simulink model "jumeau_banc_rw"  (R2025b)
settings: Solver=ode23t  StartTime=0.0  StopTime=20  MaxStep=1e-3  RelTol=1e-4
PostLoadFcn:
  | d = fileparts(get_param('jumeau_banc_rw', 'FileName')); addpath(fullfile(d, 'geometrie'), fullfile(d, 'liaison'), fullfile(d, 'pilotage')); clear d
StartFcn:
  | % Jumeau Webots : au lancement, MATLAB envoie les paramètres du Model Workspace à Webots, qui remet le banc en
  | % position de départ, puis ouvre la liaison de télémétrie et la liaison de commande (liaison/pont_banc.m).
  | if strcmp(get_param('jumeau_banc_rw/Procédé', 'LabelModeActiveChoice'), 'Webots')
  |     pont_banc('ouvrir', getVariable(get_param('jumeau_banc_rw', 'ModelWorkspace'), 'config_jumeau'));
  | end
  | pilotage_banc('depart');   % interface de pilotage : nouveau lancement
StopFcn:
  | pont_banc('fermer');
  | pilotage_banc('fin');
model workspace (MATLAB code in the model file):
  | %% Jumeau numérique du banc de stabilisation à 4 roues de réaction (version 3) : paramètres
  | % Ce code est enregistré dans le modèle (Model Explorer > jumeau_banc_rw > Model Workspace).
  | % Origine : (CAO) CAO du banc version 3, (M) mesuré sur le matériel, (F) fiche technique, (Fw) firmware,
  | % (H) hypothèse à mesurer sur le banc. Masses et inerties des pièces : dans chaque bloc de pièce.
  | 
  | %% Montage de l'essai
  | pivot_mm = 25;              % position du pivot de tangage sur le corps : 25, 24, 16, 8, 0, -8 mm (25 : banc équilibré, rangée +24 et paliers remontés de 1 mm)
  | blocage_roulis = 0;         % goupille de blocage : 1 = axe bloqué à 0°, 0 = axe libre
  | blocage_tangage = 0;
  | angle0_roulis_deg = 2;      % position de départ (mise à 0 si l'axe est bloqué)
  | angle0_tangage_deg = -1;
  | g = 9.81;                   % m/s²
  | 
  | %% Pupitre : pilotage manuel des 4 ESC
  | essai_t = 1;                % s, instant de l'échelon d'essai ajouté aux curseurs
  | essai_echelon_us = [0 0 0 0];   % µs, échelon d'essai sur chaque ESC (0 : aucun)
  | 
  | %% Alimentation des ESC
  | V_alim = 12;                % V, alimentation de labo (H : tension réglée)
  | 
  | %% ESC Brushless 30A bidirectionnels (x4)
  | f_trame_esc = 50;           % Hz, une impulsion toutes les 20 ms (Fw : LEDC 50 Hz)
  | imp_neutre = 1500;          % µs, neutre (testé sur le banc)
  | imp_min = 1000;             % µs (Fw)
  | imp_max = 2000;             % µs (Fw)
  | zone_morte_us = 0;          % µs autour du neutre (H)
  | tau_esc = 2e-3;             % s, temps de réponse de l'ESC (H)
  | armement_actif = 1;         % 1 : l'ESC ne pilote le moteur qu'après t_armement au neutre
  | t_armement = 1;             % s (H)
  | fenetre_armement_us = 25;   % µs, écart au neutre accepté pendant l'armement (H)
  | sens_moteurs = [1 1 1 1];   % +1 : au-dessus du neutre, la roue tourne dans le sens +axe (vers l'extérieur) (H : ordre des phases)
  | 
  | %% Moteurs A2212 1400 KV (x4), modèle équivalent continu
  | KV = 1400;                  % tr/min/V (F)
  | Ke = 60/(2*pi*KV);          % V.s/rad
  | Kt = Ke;                    % N.m/A
  | R_moteur = 0.08;            % ohm (H)
  | L_moteur = 30e-6;           % H (H)
  | f_roue = 5e-6;              % N.m.s/rad, frottement visqueux des roulements du moteur (H)
  | 
  | %% Cardan
  | butee_deg = 20;             % débattement de chaque axe (CAO)
  | k_butee = 20;               % N.m/rad, contact goupille-lumière (H)
  | c_butee = 0.2;              % N.m.s/rad (H)
  | b_cardan = 1e-4;            % N.m.s/rad, frottement des roulements 625 (H)
  | k_cables = 0;               % N.m/rad, raideur des deux câbles vers la table (H)
  | 
  | %% BNO055 (mode fusion)
  | T_bno = 0.01;               % s, données de fusion à 100 Hz (F)
  | bruit_bno = 1;              % 1 : bruit de mesure, 0 : capteur parfait
  | sigma_angle_deg = 0.05;     % ° (H)
  | sigma_gyro_dps = 0.1;       % °/s (H)
  | sigma_acc = 0.02;           % m/s² (H)
  | R_montage_bno = eye(3);     % axes du capteur dans le repère du dispositif : eye(3) = remappage AXIS_MAP réglé
  |                             % (la carte est tournée de 90° dans la CAO)
  | 
  | %% Capteurs de vitesse TCRT5000 (x4) : un front à chaque rayon du disque
  | n_rayons = 4;               % rayons du disque vus par tour (CAO : disque d'origine)
  | T_tcrt = 1e-3;              % s, pas de calcul du capteur (les fronts sont datés par interpolation, comme un chronomètre en µs)
  | t_arret_tcrt = 0.2;         % s sans front : la vitesse mesurée retombe à 0 (Fw, à fixer)
  | 
  | %% Pont vers le jumeau Webots (et, plus tard, vers l'ESP32 du banc réel)
  | T_pont = 0.01;              % s, une trame de commande et une trame de télémétrie toutes les 10 ms
  | 
  | %% Essai : maintien au départ et perturbation
  | t_lacher = 2;                % s, le dispositif est tenu à la main à sa position de départ jusqu'à cet instant (0 : libre dès le départ)
  | k_main = 5;                  % N.m/rad, raideur de la main qui tient le dispositif
  | c_main = 0.3;                % N.m.s/rad, son amortissement
  | perturbation_t = 7;          % s, instant de la poussée d'essai
  | perturbation_duree = 0.2;    % s
  | perturbation_couple = [0.02 0.02];   % N.m, couple de la poussée sur [roulis tangage], programmée (0 : aucune ; l'interface de pilotage en ajoute)
  | 
  | %% Grandeurs dérivées
  | assert(any(pivot_mm == [25 24 16 8 0 -8]), 'pivot_mm : 25, 24, 16, 8, 0, -8');
  | q0_deg = [angle0_roulis_deg angle0_tangage_deg] .* ([blocage_roulis blocage_tangage] == 0);
  | config_jumeau = [pivot_mm; blocage_roulis; blocage_tangage; q0_deg(:); V_alim; f_trame_esc; imp_neutre; imp_min; imp_max; ...
  |     zone_morte_us; tau_esc; armement_actif; t_armement; fenetre_armement_us; sens_moteurs(:); Ke; Kt; R_moteur; L_moteur; ...
  |     f_roue; butee_deg; k_butee; c_butee; b_cardan; k_cables; g; T_bno; bruit_bno; sigma_angle_deg; sigma_gyro_dps; ...
  |     sigma_acc; n_rayons; t_arret_tcrt; T_tcrt; R_montage_bno(:); T_pont; t_lacher; k_main; c_main];   % 51 valeurs envoyées au jumeau Webots au lancement
  | 
  | %% Commande bas niveau : une boucle de vitesse par roue, avec observateur CFO (méthode du TP2, ramenée à la vitesse)
  | J_roue = 1.562e-4;          % kg.m², inertie d'une roue autour de son axe : disque, vis, cloche du moteur (CAO)
  | T_cbn = 1/f_trame_esc;      % s, période de calcul de la commande : celle des ESC, qui ne lisent qu'une impulsion toutes les 20 ms
  | wc_roue = [10 10 10 10];    % rad/s, rapidité du suivi de vitesse de chaque roue (pôle de l'erreur en -wc)
  | wo_roue = [5 5 5 5];        % rad/s, rapidité du CFO de chaque roue (pôles en -wo et -4 wo) ; au-delà de 10, il devient instable à 20 ms
  | imp_cmd_min = 1375;         % µs, limites des impulsions commandées : vitesse conseillée des disques, 3 900 tr/min
  | imp_cmd_max = 1625;         % µs
  | w_aveugle = 45;             % rad/s, en dessous (vitesse du modèle), le TCRT5000 voit mal la roue : le CFO ne se corrige plus sur la mesure
  | 
  | %% Consigne d'essai des roues : ajoutée à la consigne qui vient de la conversion (0 tant qu'elle est vide)
  | essai_roue_t1 = 2;                  % s, départ vers le premier palier
  | essai_roue_vitesse1 = [0 0 0 0];  % rad/s, premier palier de chaque roue (0 : la roue reste à l'arrêt)
  | essai_roue_t2 = 6;                  % s, départ vers le second palier
  | essai_roue_vitesse2 = [0 0 0 0];    % rad/s, second palier de chaque roue
  | essai_roue_acc = 300;               % rad/s², pente des rampes entre les paliers
  | 
  | %% Commande bas niveau : grandeurs calculées
  | % modèle local d'une roue : d(omega)/dt = -a1 omega + a0 V + d
  | a0_roue = Kt/(R_moteur*J_roue) * [1 1 1 1];                % rad/s² par volt
  | a1_roue = (Kt*Ke/R_moteur + f_roue)/J_roue * [1 1 1 1];    % 1/s
  | K_roue = wc_roue - a1_roue;                                % retour d'état : erreur en -(a1 + K) = -wc
  | l1_roue = 5*wo_roue;                                       % CFO
  | lambda_roue = 4/5*wo_roue;
  | 
  | %% Référence : angles demandés au dispositif, en polynômes de degré 5 entre deux paliers
  | ref_t = [2 12];              % s, instant de départ vers chaque palier
  | ref_roulis_deg = [0 5];      % °, roulis demandé à chaque palier
  | ref_tangage_deg = [0 0];     % °, tangage demandé à chaque palier
  | ref_duree = 1.5;             % s, durée du passage d'un palier au suivant
  | 
  | %% Commande haut niveau : une boucle par axe [roulis tangage], placement de pôles basé sur l'observateur CFO (TP2)
  | T_chn = T_cbn;               % s, période de calcul : celle de la commande bas niveau et des ESC
  | t_depart = t_lacher;         % s, mise en marche de la commande : au moment où la main lâche le dispositif
  | wc_axe = [4 4];              % rad/s, rapidité du suivi d'angle de chaque axe
  | xi_axe = [1 1];              % amortissement
  | wo_axe = [3 3];              % rad/s, rapidité du CFO de chaque axe (pôles en -wo et -4 wo, double) ; au-delà de 4, le couple s'agite
  | desat_active = 0;            % 1 : la référence est décalée pour ramener les roues vers leur vitesse de repos
  | T_desat = 5;                 % s, constante de temps de ce retour
  | desat_max_deg = 15;          % °, décalage maximal de la référence
  | 
  | %% Conversion : couples des deux axes vers les 4 roues
  | w_repos = 200;               % rad/s, vitesse de repos des 4 roues : elles tournent toujours, le TCRT5000 les voit toujours
  | t_roues = t_armement + 0.2;  % s, mise en rotation des roues, une fois les ESC armés
  | acc_roue_max = 300;          % rad/s², accélération maximale demandée à une roue
  | w_roue_min = 60;             % rad/s, vitesses limites demandées à une roue
  | w_roue_max = 400;            % rad/s (disques : 3 900 tr/min conseillés, soit 408 rad/s)
  | 
  | %% Masses et inerties utilisées par la commande (CAO du banc version 3)
  | m_disp = 1.2615;             % kg, dispositif et ses 4 roues
  | zG_disp = 24.977e-3;         % m, hauteur de son centre de masse sur le corps (le pivot est à pivot_mm)
  | Ixx_disp_24 = 8.2684e-3;     % kg.m², inertie du dispositif autour du roulis, pivot à +24 mm
  | Iyy_disp_24 = 8.2786e-3;     % kg.m², autour du tangage, pivot à +24 mm
  | m_croix = 0.0755;            % kg, croisillon et paliers (ne tournent qu'en roulis)
  | zG_croix = 0.257e-3;         % m, hauteur de leur centre de masse au-dessus de l'axe de roulis
  | Ixx_croix = 2.073e-4;        % kg.m²
  | 
  | %% Commande haut niveau et conversion : grandeurs calculées
  | % modèle local d'un axe : d²(theta)/dt² = -a1 d(theta)/dt + a0 C + d, avec C le couple demandé aux roues
  | hz = zG_disp - pivot_mm/1000;                                    % m, centre de masse du dispositif au-dessus du pivot
  | I_axe = [Ixx_disp_24 + Ixx_croix, Iyy_disp_24] + m_disp*(hz^2 - (zG_disp - 0.024)^2) - 2*J_roue;   % kg.m²
  | mgh_axe = g*[m_disp*hz + m_croix*zG_croix, m_disp*hz];           % N.m/rad, couple de pesanteur par radian d'inclinaison
  | a0_axe = 1./I_axe;                                               % rad/s² par N.m
  | a1_axe = b_cardan./I_axe;                                        % 1/s
  | k1_axe = wc_axe.^2;                                              % retour d'état : s² + 2 xi wc s + wc²
  | k2_axe = 2*xi_axe.*wc_axe - a1_axe;
  | l1_axe = 9*wo_axe;                                               % CFO du TP2
  | l2_axe = 12*wo_axe.^2;
  | lambda_axe = 4/3*wo_axe;
  | C_max = 2*J_roue*cosd(45)*acc_roue_max;                          % N.m, couple maximal demandé sur un axe
  | k_desat = desat_active.*sign(mgh_axe + (mgh_axe == 0))./(max(abs(mgh_axe), 1e-3)*T_desat);            % rad par N.m.s
  | sx_roues = [1 -1 -1 1];                                          % signe de cos(45°, 135°, 225°, 315°) : part de chaque roue sur le roulis
  | sy_roues = [1 1 -1 -1];                                          % signe de sin : part sur le tangage
  | M_conv = -[sx_roues(:) sy_roues(:)]/(4*J_roue*cosd(45));         % accélération des 4 roues pour un couple [roulis; tangage]
  | 
  | %% Perception : des mesures à l'état du banc
  | T_perception = T_bno;        % s, période de calcul : celle du BNO055
  | tau_desequilibre = 2;        % s, constante de temps du filtre du couple extérieur et du déséquilibre
  | 
  | %% Pilotage par l'interface (pilotage/pilote_banc.m)
  | manche_max_deg = 15;         % °, limite de sécurité de l'inclinaison demandée par le manche (l'interface règle l'amplitude)
  | w_manche = 3;                % rad/s, rapidité avec laquelle la référence rejoint le manche (second ordre critique)
  | T_affichage = 0.1;           % s, rafraîchissement de l'interface
undefined symbols (not defined in the file): DiscIntNeverNeededParam, X, Y, Z
libraries: sm_lib x256, nesl_utility x24, simulink x7
(part 1 of 8)
CloseFcn:
  | try, d = fileparts(get_param('jumeau_banc_rw', 'FileName')); rmpath(fullfile(d, 'geometrie'), fullfile(d, 'liaison'), fullfile(d, 'pilotage')); clear d, catch, end
settings Model: Creator=FOFIEVIGOLBRYAN  LastModifiedBy=FOFIEVIGOLBRYAN

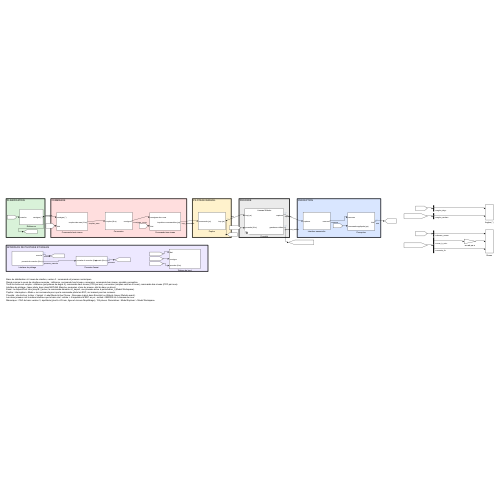
[thumbnail: Simulink's stored preview of the top-level diagram]
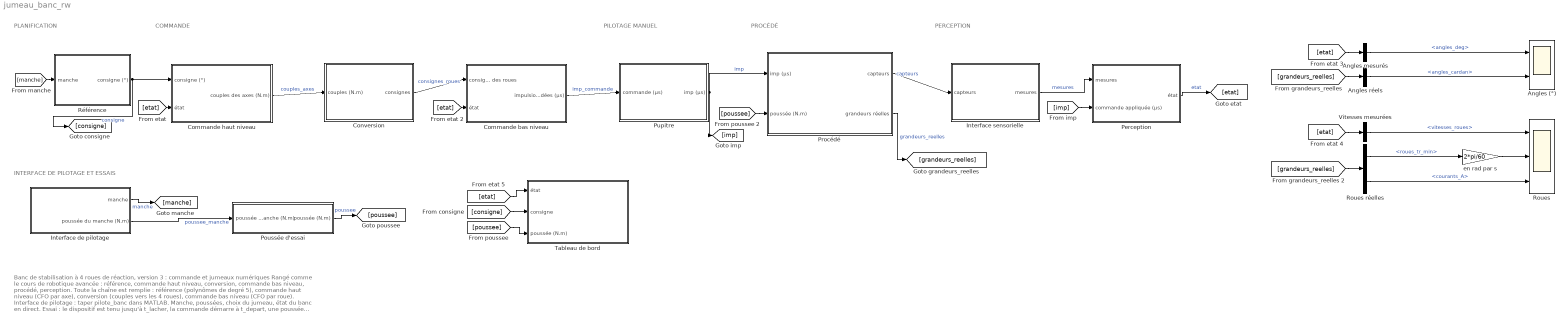
== system jumeau_banc_rw ==
  note: PLANIFICATION
  note: COMMANDE
  note: PILOTAGE MANUEL
  note: PROCÉDÉ
  note: PERCEPTION
  note: Banc de stabilisation à 4 roues de réaction, version 3 : commande et jumeaux numériques
      | Rangé comme le cours de robotique avancée : référence, commande haut niveau, conversion, commande bas niveau, procédé, perception.
      | Toute la chaîne est remplie : référence (polynômes de degré 5), commande haut niveau (CFO par axe), conversion (couples vers les 4 roues), commande bas niveau (CFO par roue).
      | Interface de pilotage : taper pilote_banc dans MATLAB. Manche, poussées, choix du jumeau, état du banc en direct.
      | Essai : le dispositif est tenu jusqu'à t_lacher, la commande démarre à t_depart, une poussée arrive à perturbation_t (Model Workspace).
      | Pupitre : interrupteur « Mode » sur commande pour que la commande pilote les ESC, sur manuel pour les curseurs.
      | Procédé : clic droit sur le bloc > Variant > Label Mode Active Choice : Simscape (calcul dans Simulink) ou Webots (lancer Webots avant).
      | Les deux jumeaux ont la même interface que le banc réel : entrée = 4 impulsions d'ESC en µs ; sorties = BNO055 et 4 vitesses de roue.
      | Mécanique : CAO du banc version 3, équilibrée (pivot à +25 mm, tiges et écrous d'équilibrage), 124 pièces. Paramètres : Model Explorer > Model Workspace.
  note: INTERFACE DE PILOTAGE ET ESSAIS
  Angles (°) : Scope  NumInputPorts=2
      settings: Title=cardan réel : roulis, tangage (°)
  Angles mesurés : BusSelector  OutputSignals=angles_deg
  Angles réels : BusSelector  OutputSignals=angles_cardan
  Commande bas niveau : Subsystem  Description=Commande bas niveau : boucle de vitesse de chaque roue par placement de pôles basé sur l'observateur CFO.
  Commande haut niveau : Subsystem  Description=Commande haut niveau : stabilisation de l'inclinaison par placement de pôles basé sur l'observateur CFO, une boucle par axe.
  Conversion : Subsystem  Description=Conversion : couples des deux axes vers vitesse et accélération de chaque roue.
  Interface de pilotage : Subsystem  Description=Lit le manche et les poussées de l'interface de pilotage.
  Interface sensorielle : Subsystem
  Perception : Subsystem  Description=Perception : des mesures du banc (BNO055, TCRT5000, impulsions envoyées) à son état.
  Poussée d'essai : Subsystem  Description=Poussée d'essai : programmée et demandée par l'interface, envoyée au procédé.
  Procédé : Subsystem  Variant=on  VariantControlMode=label  LabelModeActiveChoice=Webots
  Pupitre : Subsystem
  Roues : Scope  NumInputPorts=3
      settings: ActiveDisplayString=3  Title=courant des moteurs (A)  ActiveDisplayYMinimum=-1  ActiveDisplayYMaximum=1
  Roues réelles : BusSelector  OutputSignals=roues_tr_min,courants_A
  Référence : Subsystem  Description=Référence : angles demandés au dispositif, programmés ou donnés par le manche de l'interface de pilotage.
  Tableau de bord : Subsystem  Description=Tableau de bord : envoie l'état du banc à l'interface de pilotage.
  Vitesses mesurées : BusSelector  OutputSignals=vitesses_roues
  en rad par s : Gain  Gain=2*pi/60
  wires:
  Référence/1(consigne (°)) -> Commande haut niveau/1(consigne (°)), [consigne]  "consigne"
  Commande haut niveau/1(couples des axes (N.m)) -> Conversion/1(couples (N.m))  "couples_axes"
  Conversion/1(consignes) -> Commande bas niveau/1(consignes des roues)  "consignes_roues"
  Commande bas niveau/1(impulsions commandées (µs)) -> Pupitre/1(commande (µs))  "imp_commande"
  Pupitre/1(imp (µs)) -> Procédé/1(imp (µs)), [imp]  "imp"
  Procédé/1(capteurs) -> Interface sensorielle/1(capteurs)  "capteurs"
  Interface sensorielle/1(mesures) -> Perception/1(mesures)  "mesures"
  Perception/1(état) -> [etat]  "etat"
  [etat] -> Commande haut niveau/2(état)
  [etat] -> Commande bas niveau/2(état)
  Procédé/2(grandeurs réelles) -> [grandeurs_reelles]  "grandeurs_reelles"
  [etat] -> Angles mesurés/1
  [grandeurs_reelles] -> Angles réels/1
  [etat] -> Vitesses mesurées/1
  [grandeurs_reelles] -> Roues réelles/1
  Angles mesurés/1 -> Angles (°)/1  "<angles_deg>"
  Angles réels/1 -> Angles (°)/2  "<angles_cardan>"
  Vitesses mesurées/1 -> Roues/1  "<vitesses_roues>"
  Roues réelles/1 -> en rad par s/1  "<roues_tr_min>"
  en rad par s/1 -> Roues/2
  Roues réelles/2 -> Roues/3  "<courants_A>"
  [imp] -> Perception/2(commande appliquée (µs))
  [manche] -> Référence/1(manche)
  Interface de pilotage/1(manche) -> [manche]  "manche"
  Interface de pilotage/2(poussée du manche (N.m)) -> Poussée d'essai/1(poussée du manche (N.m))  "poussee_manche"
  Poussée d'essai/1(poussée (N.m)) -> [poussee]  "poussee"
  [etat] -> Tableau de bord/1(état)
  [consigne] -> Tableau de bord/2(consigne)
  [poussee] -> Tableau de bord/3(poussée (N.m))
  [poussee] -> Procédé/2(poussée (N.m))

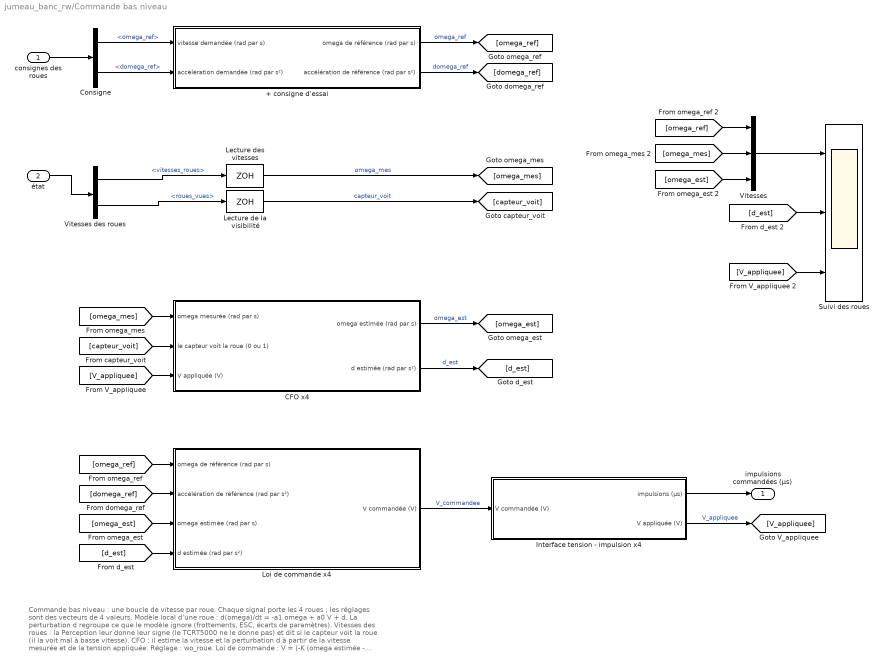
== system jumeau_banc_rw/Commande bas niveau ==
  note: Commande bas niveau : une boucle de vitesse par roue. Chaque signal porte les 4 roues ; les réglages sont des vecteurs de 4 valeurs.
      | Modèle local d'une roue : d(omega)/dt = -a1 omega + a0 V + d. La perturbation d regroupe ce que le modèle ignore (frottements, ESC, écarts de paramètres).
      | Vitesses des roues : la Perception leur donne leur signe (le TCRT5000 ne le donne pas) et dit si le capteur voit la roue (il la voit mal à basse vitesse).
      | CFO : il estime la vitesse et la perturbation d à partir de la vitesse mesurée et de la tension appliquée. Réglage : wo_roue.
      | Loi de commande : V = (-K (omega estimée - omega de référence) - d estimée + a1 omega de référence + accélération de référence) / a0. Réglage : wc_roue.
      | Interface : la tension devient une impulsion d'ESC, bornée de imp_cmd_min à imp_cmd_max. Le CFO reçoit la tension réellement appliquée.
      | Consigne d'essai : essai_roue_... dans le Model Workspace. Pour que la commande pilote les ESC : interrupteur « Mode » du Pupitre sur commande.
  consignes des roues : Inport
  état : Inport  Port=2
  + consigne d'essai : Subsystem
  CFO x4 : Subsystem
  Consigne : BusSelector  OutputSignals=omega_ref,domega_ref
  Interface tension - impulsion x4 : Subsystem
  Lecture de la visibilité : ZeroOrderHold  SampleTime=T_cbn
  Lecture des vitesses : ZeroOrderHold  SampleTime=T_cbn
  Loi de commande x4 : Subsystem
  Suivi des roues : Scope  NumInputPorts=3
      settings: ActiveDisplayString=3  Title=tension appliquée aux moteurs (V)
  Vitesses : Mux  Inputs=3
  Vitesses des roues : BusSelector  OutputSignals=vitesses_roues,roues_vues
  impulsions commandées (µs) : Outport
  wires:
  consignes des roues/1 -> Consigne/1
  Consigne/1 -> + consigne d'essai/1(vitesse demandée (rad par s))  "<omega_ref>"
  Consigne/2 -> + consigne d'essai/2(accélération demandée (rad par s²))  "<domega_ref>"
  + consigne d'essai/1(omega de référence (rad par s)) -> [omega_ref]  "omega_ref"
  + consigne d'essai/2(accélération de référence (rad par s²)) -> [domega_ref]  "domega_ref"
  état/1 -> Vitesses des roues/1
  Vitesses des roues/1 -> Lecture des vitesses/1  "<vitesses_roues>"
  Vitesses des roues/2 -> Lecture de la visibilité/1  "<roues_vues>"
  Lecture des vitesses/1 -> [omega_mes]  "omega_mes"
  Lecture de la visibilité/1 -> [capteur_voit]  "capteur_voit"
  [omega_mes] -> CFO x4/1(omega mesurée (rad par s))
  [capteur_voit] -> CFO x4/2(le capteur voit la roue (0 ou 1))
  [V_appliquee] -> CFO x4/3(V appliquée (V))
  CFO x4/1(omega estimée (rad par s)) -> [omega_est]  "omega_est"
  CFO x4/2(d estimée (rad par s²)) -> [d_est]  "d_est"
  [omega_ref] -> Loi de commande x4/1(omega de référence (rad par s))
  [domega_ref] -> Loi de commande x4/2(accélération de référence (rad par s²))
  [omega_est] -> Loi de commande x4/3(omega estimée (rad par s))
  [d_est] -> Loi de commande x4/4(d estimée (rad par s²))
  Loi de commande x4/1(V commandée (V)) -> Interface tension - impulsion x4/1(V commandée (V))  "V_commandee"
  Interface tension - impulsion x4/1(impulsions (µs)) -> impulsions commandées (µs)/1
  Interface tension - impulsion x4/2(V appliquée (V)) -> [V_appliquee]  "V_appliquee"
  [omega_ref] -> Vitesses/1
  [omega_mes] -> Vitesses/2
  [omega_est] -> Vitesses/3
  Vitesses/1 -> Suivi des roues/1
  [d_est] -> Suivi des roues/2
  [V_appliquee] -> Suivi des roues/3

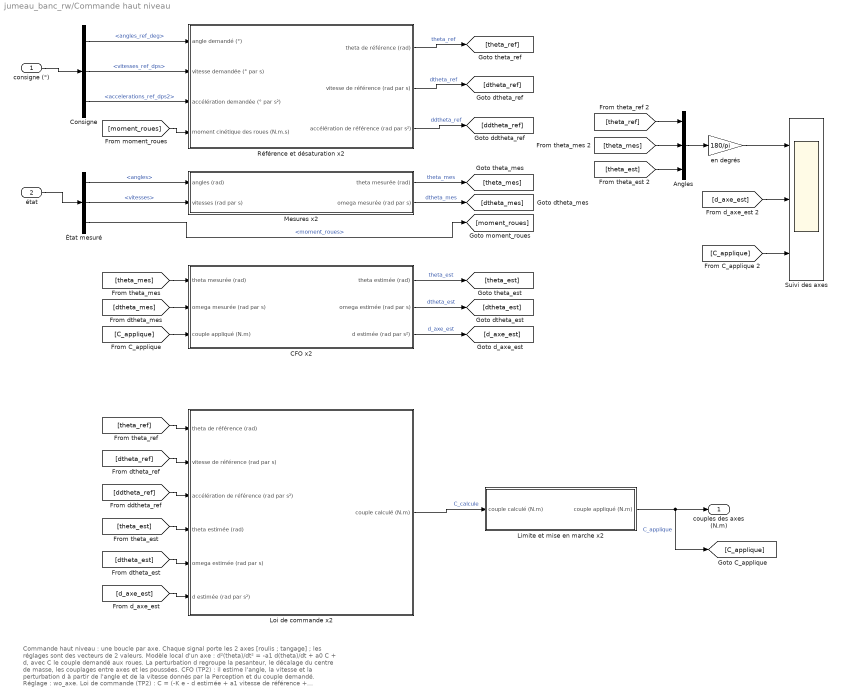
== system jumeau_banc_rw/Commande haut niveau ==
  note: Commande haut niveau : une boucle par axe. Chaque signal porte les 2 axes [roulis ; tangage] ; les réglages sont des vecteurs de 2 valeurs.
      | Modèle local d'un axe : d²(theta)/dt² = -a1 d(theta)/dt + a0 C + d, avec C le couple demandé aux roues. La perturbation d regroupe la pesanteur,
      | le décalage du centre de masse, les couplages entre axes et les poussées.
      | CFO (TP2) : il estime l'angle, la vitesse et la perturbation d à partir de l'angle et de la vitesse donnés par la Perception et du couple demandé. Réglage : wo_axe.
      | Loi de commande (TP2) : C = (-K e - d estimée + a1 vitesse de référence + accélération de référence) / a0. Réglages : wc_axe, xi_axe.
      | Désaturation : la référence est décalée pour que la pesanteur ramène les roues à leur vitesse de repos. Réglages : desat_active, T_desat.
      | La commande démarre à t_depart, quand la main lâche le dispositif. Le couple est borné à C_max.
  consigne (°) : Inport
  état : Inport  Port=2
  Angles : Mux  Inputs=3
  CFO x2 : Subsystem
  Consigne : BusSelector  OutputSignals=angles_ref_deg,vitesses_ref_dps,accelerations_ref_dps2
  Limite et mise en marche x2 : Subsystem
  Loi de commande x2 : Subsystem
  Mesures x2 : Subsystem
  Référence et désaturation x2 : Subsystem
  Suivi des axes : Scope  NumInputPorts=3
      settings: ActiveDisplayString=3  Title=couples demandés aux roues (N.m)
  en degrés : Gain  Gain=180/pi
  État mesuré : BusSelector  OutputSignals=angles,vitesses,moment_roues
  couples des axes (N.m) : Outport
  wires:
  consigne (°)/1 -> Consigne/1
  Consigne/1 -> Référence et désaturation x2/1(angle demandé (°))  "<angles_ref_deg>"
  Consigne/2 -> Référence et désaturation x2/2(vitesse demandée (° par s))  "<vitesses_ref_dps>"
  Consigne/3 -> Référence et désaturation x2/3(accélération demandée (° par s²))  "<accelerations_ref_dps2>"
  [moment_roues] -> Référence et désaturation x2/4(moment cinétique des roues (N.m.s))
  Référence et désaturation x2/1(theta de référence (rad)) -> [theta_ref]  "theta_ref"
  Référence et désaturation x2/2(vitesse de référence (rad par s)) -> [dtheta_ref]  "dtheta_ref"
  Référence et désaturation x2/3(accélération de référence (rad par s²)) -> [ddtheta_ref]  "ddtheta_ref"
  état/1 -> État mesuré/1
  État mesuré/1 -> Mesures x2/1(angles (rad))  "<angles>"
  État mesuré/2 -> Mesures x2/2(vitesses (rad par s))  "<vitesses>"
  État mesuré/3 -> [moment_roues]  "<moment_roues>"
  Mesures x2/1(theta mesurée (rad)) -> [theta_mes]  "theta_mes"
  Mesures x2/2(omega mesurée (rad par s)) -> [dtheta_mes]  "dtheta_mes"
  [theta_mes] -> CFO x2/1(theta mesurée (rad))
  [dtheta_mes] -> CFO x2/2(omega mesurée (rad par s))
  [C_applique] -> CFO x2/3(couple appliqué (N.m))
  CFO x2/1(theta estimée (rad)) -> [theta_est]  "theta_est"
  CFO x2/2(omega estimée (rad par s)) -> [dtheta_est]  "dtheta_est"
  CFO x2/3(d estimée (rad par s²)) -> [d_axe_est]  "d_axe_est"
  [theta_ref] -> Loi de commande x2/1(theta de référence (rad))
  [dtheta_ref] -> Loi de commande x2/2(vitesse de référence (rad par s))
  [ddtheta_ref] -> Loi de commande x2/3(accélération de référence (rad par s²))
  [theta_est] -> Loi de commande x2/4(theta estimée (rad))
  [dtheta_est] -> Loi de commande x2/5(omega estimée (rad par s))
  [d_axe_est] -> Loi de commande x2/6(d estimée (rad par s²))
  Loi de commande x2/1(couple calculé (N.m)) -> Limite et mise en marche x2/1(couple calculé (N.m))  "C_calcule"
  Limite et mise en marche x2/1(couple appliqué (N.m)) -> couples des axes (N.m)/1, [C_applique]  "C_applique"
  [theta_ref] -> Angles/1
  [theta_mes] -> Angles/2
  [theta_est] -> Angles/3
  Angles/1 -> en degrés/1
  en degrés/1 -> Suivi des axes/1
  [d_axe_est] -> Suivi des axes/2
  [C_applique] -> Suivi des axes/3

== system jumeau_banc_rw/Conversion ==
  note: Conversion : couples demandés sur les deux axes vers la vitesse et l'accélération de chaque roue.
      | Une roue qui accélère pousse le dispositif en sens inverse : accélération des 4 roues = M_conv [couple de roulis ; couple de tangage].
      | Les roues sont à 45°, 135°, 225° et 315° : chacune agit sur les deux axes, à part égale (cos 45°).
      | L'accélération s'ajoute à la vitesse de repos w_repos, la même pour les 4 roues : deux roues opposées tournent alors en sens contraire
      | et leurs effets s'annulent. Les roues ne passent jamais par l'arrêt, où le TCRT5000 ne les voit plus.
      | Limites : acc_roue_max sur l'accélération, w_roue_min et w_roue_max sur la vitesse demandée.
  couples (N.m) : Inport
  Accélération demandée : Sum
  Accélération maximale : Saturate  UpperLimit=acc_roue_max  LowerLimit=-acc_roue_max
  Consignes : BusCreator  Description=omega_ref : vitesse demandée à chaque roue (rad/s). domega_ref : son accélération (rad/s²).  Inputs=2
  Mise en rotation : Step  Time=t_roues  Before=[0; 0; 0; 0]  After=w_repos*[1; 1; 1; 1]  SampleTime=T_chn
  Pente de la rampe : simulink/Discrete/Discrete Derivative  gainval=1.0  ICPrevScaledInput=0.0  OutMin=[]  OutMax=[]  OutDataType=fixdt(1, 16)  OutScaling=2^-10  DoSatur=off
  Rampe : RateLimiter  RisingSlewLimit=acc_roue_max  FallingSlewLimit=-acc_roue_max  SampleTimeMode=inherited
  Répartition sur les 4 roues : Gain  Gain=M_conv  Multiplication=Matrix(K*u)
  Vitesse demandée : Sum
  Écart à la vitesse de repos : DiscreteIntegrator  gainval=1  SampleTime=T_chn  LimitOutput=on  UpperSaturationLimit=max(w_roue_max - w_repos, 0)  LowerSaturationLimit=min(w_roue_min - w_repos, 0)  ICPrevOutput=DiscIntNeverNeededParam  ICPrevScaledInput=DiscIntNeverNeededParam
  consignes : Outport
  wires:
  couples (N.m)/1 -> Répartition sur les 4 roues/1
  Répartition sur les 4 roues/1 -> Accélération maximale/1
  Accélération maximale/1 -> [acceleration]  "acceleration"
  [acceleration] -> Écart à la vitesse de repos/1
  Écart à la vitesse de repos/1 -> [ecart_vitesse]  "ecart_vitesse"
  Mise en rotation/1 -> Rampe/1
  Rampe/1 -> [vitesse_repos], Pente de la rampe/1  "vitesse_repos"
  Pente de la rampe/1 -> [acceleration_repos]  "acceleration_repos"
  [ecart_vitesse] -> Vitesse demandée/1
  [vitesse_repos] -> Vitesse demandée/2
  [acceleration] -> Accélération demandée/1
  [acceleration_repos] -> Accélération demandée/2
  Vitesse demandée/1 -> Consignes/1  "omega_ref"
  Accélération demandée/1 -> Consignes/2  "domega_ref"
  Consignes/1 -> consignes/1

== system jumeau_banc_rw/Interface de pilotage ==
  note: Lit l'interface de pilotage (pilotage/pilote_banc.m, échange par pilotage/pilotage_banc.m) à chaque période de la commande.
      | manche = [actif ; roulis demandé ; tangage demandé] (°) ; poussée en cours sur [roulis ; tangage] (N.m).
      | Interface fermée : le manche est inactif (la référence programmée s'applique) et il n'y a aucune poussée.
  Lecture de l'interface : MATLAB Function  TreatAsAtomicUnit=on
  Temps : DigitalClock  SampleTime=T_chn
  manche : Outport
  poussée du manche (N.m) : Outport  Port=2
  wires:
  Temps/1 -> Lecture de l'interface/1(t)
  Lecture de l'interface/1(manche) -> manche/1
  Lecture de l'interface/2(poussee) -> poussée du manche (N.m)/1

== system jumeau_banc_rw/Interface sensorielle ==
  note: Interface sensorielle : ce que l'ESP32 lit sur les capteurs, mis en grandeurs utiles.
      | BNO055 : euler = [cap ; roulis ; tangage] en degrés, gyroscope en °/s. TCRT5000 : vitesse de chaque roue, sans signe.
  note: Quaternion : l'orientation du capteur, au pas de 2^-14. La Perception en tire des angles 8 fois plus fins que les angles d'Euler.
  capteurs : Inport
  Gyroscope : SignalConversion  OverrideOpt=off
  Mesures : BusCreator  Description=angles_deg = [roulis; tangage] (°, angles d'Euler), gyro_dps (°/s, axes du capteur), vitesses_roues (rad/s, sans signe), quaternion [w; x; y; z] (orientation du capteur).  Inputs=4
  Quaternion : SignalConversion  OverrideOpt=off
  Registres lus : BusSelector  OutputSignals=BNO055.euler,BNO055.gyro,vitesses_roues,BNO055.quat
  "Roulis, tangage" : Selector  InputPortWidth=3  IndexOptions=Index vector (dialog)  Indices=[2 3]  OutputSizes=1
  mesures : Outport
  wires:
  capteurs/1 -> Registres lus/1
  Registres lus/1 -> "Roulis, tangage"/1  "<euler>"
  "Roulis, tangage"/1 -> Mesures/1  "angles_deg"
  Registres lus/2 -> Gyroscope/1  "<gyro>"
  Gyroscope/1 -> Mesures/2  "gyro_dps"
  Registres lus/3 -> Mesures/3  "<vitesses_roues>"
  Mesures/1 -> mesures/1
  Registres lus/4 -> Quaternion/1  "<quat>"
  Quaternion/1 -> Mesures/4  "quaternion"

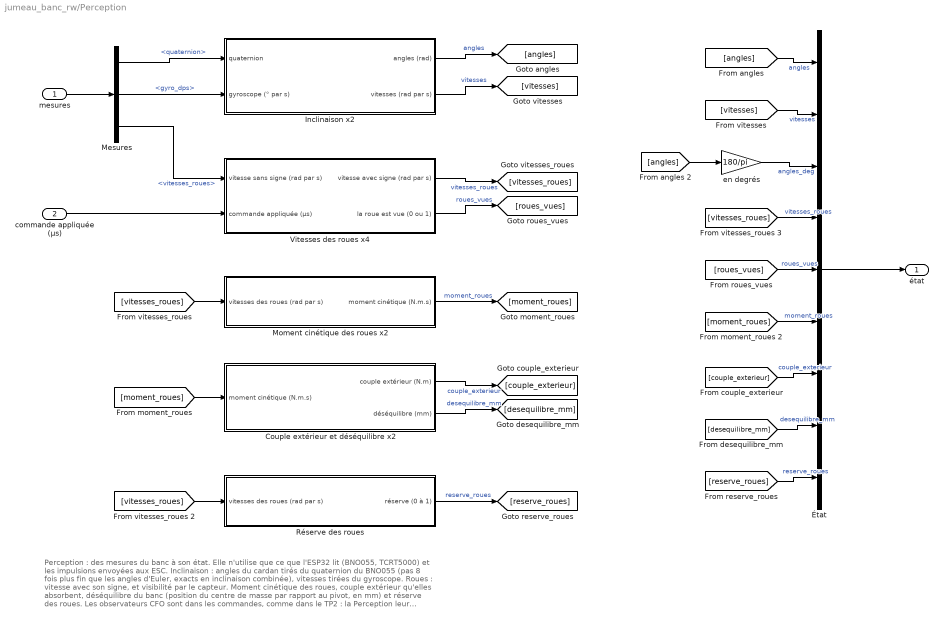
== system jumeau_banc_rw/Perception ==
  note: Perception : des mesures du banc à son état. Elle n'utilise que ce que l'ESP32 lit (BNO055, TCRT5000) et les impulsions envoyées aux ESC.
      | Inclinaison : angles du cardan tirés du quaternion du BNO055 (pas 8 fois plus fin que les angles d'Euler, exacts en inclinaison combinée),
      | vitesses tirées du gyroscope. Roues : vitesse avec son signe, et visibilité par le capteur. Moment cinétique des roues, couple extérieur
      | qu'elles absorbent, déséquilibre du banc (position du centre de masse par rapport au pivot, en mm) et réserve des roues.
      | Les observateurs CFO sont dans les commandes, comme dans le TP2 : la Perception leur donne des mesures propres.
  mesures : Inport
  commande appliquée (µs) : Inport  Port=2
  Couple extérieur et déséquilibre x2 : Subsystem
  Inclinaison x2 : Subsystem
  Mesures : BusSelector  OutputSignals=quaternion,gyro_dps,vitesses_roues
  Moment cinétique des roues x2 : Subsystem
  Réserve des roues : Subsystem
  Vitesses des roues x4 : Subsystem
  en degrés : Gain  Gain=180/pi
  État : BusCreator  Description=angles (rad) et angles_deg (°) : [roulis ; tangage] du cardan ; vitesses (rad/s) ; vitesses_roues (rad/s, avec signe) ; roues_vues (0 ou 1) ; moment_roues (N.m.s, sur [roulis ; tangage]) ; couple_exterieur (N.m) ; desequilibre_mm : position du centre de masse par rapport au pivot, [selon X ; selon Y] ; reserve_roues (0 à 1).  Inputs=9
  état : Outport
  wires:
  mesures/1 -> Mesures/1
  Mesures/1 -> Inclinaison x2/1(quaternion)  "<quaternion>"
  Mesures/2 -> Inclinaison x2/2(gyroscope (° par s))  "<gyro_dps>"
  Inclinaison x2/1(angles (rad)) -> [angles]  "angles"
  Inclinaison x2/2(vitesses (rad par s)) -> [vitesses]  "vitesses"
  Mesures/3 -> Vitesses des roues x4/1(vitesse sans signe (rad par s))  "<vitesses_roues>"
  commande appliquée (µs)/1 -> Vitesses des roues x4/2(commande appliquée (µs))
  Vitesses des roues x4/1(vitesse avec signe (rad par s)) -> [vitesses_roues]  "vitesses_roues"
  Vitesses des roues x4/2(la roue est vue (0 ou 1)) -> [roues_vues]  "roues_vues"
  [vitesses_roues] -> Moment cinétique des roues x2/1(vitesses des roues (rad par s))
  Moment cinétique des roues x2/1(moment cinétique (N.m.s)) -> [moment_roues]  "moment_roues"
  [moment_roues] -> Couple extérieur et déséquilibre x2/1(moment cinétique (N.m.s))
  Couple extérieur et déséquilibre x2/1(couple extérieur (N.m)) -> [couple_exterieur]  "couple_exterieur"
  Couple extérieur et déséquilibre x2/2(déséquilibre (mm)) -> [desequilibre_mm]  "desequilibre_mm"
  [vitesses_roues] -> Réserve des roues/1(vitesses des roues (rad par s))
  Réserve des roues/1(réserve (0 à 1)) -> [reserve_roues]  "reserve_roues"
  [angles] -> État/1  "angles"
  [vitesses] -> État/2  "vitesses"
  [angles] -> en degrés/1
  en degrés/1 -> État/3  "angles_deg"
  [vitesses_roues] -> État/4  "vitesses_roues"
  [roues_vues] -> État/5  "roues_vues"
  [moment_roues] -> État/6  "moment_roues"
  [couple_exterieur] -> État/7  "couple_exterieur"
  [desequilibre_mm] -> État/8  "desequilibre_mm"
  [reserve_roues] -> État/9  "reserve_roues"
  État/1 -> état/1

== system jumeau_banc_rw/Poussée d'essai ==
  note: Poussée sur [roulis ; tangage] (N.m), envoyée au procédé : la poussée programmée (perturbation_t, perturbation_duree,
      | perturbation_couple) plus les poussées demandées par l'interface de pilotage. Le banc réel l'ignorera : on le pousse avec le doigt.
  poussée du manche (N.m) : Inport
  Début de la poussée programmée : Step  Time=perturbation_t  Before=[0; 0]  After=perturbation_couple(:)  SampleTime=0
  Fin de la poussée programmée : Step  Time=perturbation_t + perturbation_duree  Before=[0; 0]  After=-perturbation_couple(:)  SampleTime=0
  Poussée : Sum  Inputs=+++
  poussée (N.m) : Outport
  wires:
  Début de la poussée programmée/1 -> Poussée/1
  Fin de la poussée programmée/1 -> Poussée/2
  poussée du manche (N.m)/1 -> Poussée/3
  Poussée/1 -> poussée (N.m)/1

== system jumeau_banc_rw/Procédé ==
  note: 1) Add Subsystem or Model blocks as valid variant choices.
      | 2) You cannot connect blocks at this level. At simulation, connectivity is automatically
      | determined, based on the active variant and port name matching.
  imp (µs) : Inport
  poussée (N.m) : Inport  Port=2
  Jumeau Simscape : Subsystem  VariantControl=Simscape
  Jumeau Webots : Subsystem  VariantControl=Webots
  capteurs : Outport
  grandeurs réelles : Outport  Port=2

== system jumeau_banc_rw/Pupitre ==
  note: Pupitre : pilotage manuel des 4 ESC, en attendant la commande.
      | Double-clic sur un curseur ESC k : impulsion de 1300 à 1700 µs (1500 = neutre). Les ESC s'arment après 1 s au neutre.
      | Échelon d'essai : essai_echelon_us (Model Workspace) s'ajoute aux curseurs à t = essai_t, pour des essais reproductibles.
      | Double-clic sur un interrupteur pour le basculer : manuel ou commande ; marche ou arrêt (neutre).
  commande (µs) : Inport
  Curseurs : Mux
  Curseurs + essai : Sum
  ESC 1 (µs) : simulink/Math Operations/Slider Gain  gain=1500  low=1300  high=1700
  ESC 2 (µs) : simulink/Math Operations/Slider Gain  gain=1500  low=1300  high=1700
  ESC 3 (µs) : simulink/Math Operations/Slider Gain  gain=1500  low=1300  high=1700
  ESC 4 (µs) : simulink/Math Operations/Slider Gain  gain=1500  low=1300  high=1700
  Marche (haut) ou arrêt (bas) : ManualSwitch
  "Mode : manuel (haut) ou commande (bas)" : ManualSwitch  CurrentSetting=0
  Neutre : Constant  Value=imp_neutre * [1; 1; 1; 1]
  un : Constant
  Échelon d'essai : Step  Time=essai_t  Before=[0; 0; 0; 0]  After=essai_echelon_us(:)  SampleTime=0
  imp (µs) : Outport
  wires:
  un/1 -> ESC 3 (µs)/1, ESC 4 (µs)/1, ESC 1 (µs)/1, ESC 2 (µs)/1
  ESC 1 (µs)/1 -> Curseurs/1
  ESC 2 (µs)/1 -> Curseurs/2
  ESC 3 (µs)/1 -> Curseurs/3
  ESC 4 (µs)/1 -> Curseurs/4
  Curseurs/1 -> Curseurs + essai/1
  Échelon d'essai/1 -> Curseurs + essai/2
  commande (µs)/1 -> [commande]  "commande"
  Curseurs + essai/1 -> "Mode : manuel (haut) ou commande (bas)"/1
  [commande] -> "Mode : manuel (haut) ou commande (bas)"/2
  "Mode : manuel (haut) ou commande (bas)"/1 -> Marche (haut) ou arrêt (bas)/1
  Neutre/1 -> Marche (haut) ou arrêt (bas)/2
  Marche (haut) ou arrêt (bas)/1 -> imp (µs)/1

== system jumeau_banc_rw/Référence ==
  note: Référence : angles de roulis et de tangage demandés au dispositif, avec leur vitesse et leur accélération.
      | Programme : à chaque instant ref_t(i), départ vers le palier [ref_roulis_deg(i) ; ref_tangage_deg(i)], atteint en ref_duree par un polynôme de degré 5.
      | Manche : quand l'interface de pilotage (pilotage/pilote_banc.m) est ouverte, l'angle vient du manche, suivi par un second ordre critique (w_manche).
      | Réglages dans le Model Workspace : ref_t, ref_roulis_deg, ref_tangage_deg, ref_duree, w_manche, manche_max_deg.
  manche : Inport
  "Choix : accélération" : Switch  Criteria=u2 > Threshold  Threshold=0.5  SaturateOnIntegerOverflow=off  InputSameDT=off
  "Choix : angle" : Switch  Criteria=u2 > Threshold  Threshold=0.5  SaturateOnIntegerOverflow=off  InputSameDT=off
  "Choix : vitesse" : Switch  Criteria=u2 > Threshold  Threshold=0.5  SaturateOnIntegerOverflow=off  InputSameDT=off
  Consigne : BusCreator  Description=angles_ref_deg (°), vitesses_ref_dps (°/s), accelerations_ref_dps2 (°/s²), [roulis ; tangage].  Inputs=3
  "Manche : filtre du second ordre" : MATLAB Function  TreatAsAtomicUnit=on
  "Programme : polynômes de degré 5" : MATLAB Function  TreatAsAtomicUnit=on
  Temps : DigitalClock  SampleTime=T_chn
  consigne (°) : Outport
  wires:
  Temps/1 -> "Programme : polynômes de degré 5"/1(t), "Manche : filtre du second ordre"/3(t)
  manche/1 -> "Manche : filtre du second ordre"/1(manche)
  "Programme : polynômes de degré 5"/1(angle) -> "Manche : filtre du second ordre"/2(angle_programme), "Choix : angle"/3
  [manche_actif] -> "Choix : angle"/2
  [manche_actif] -> "Choix : vitesse"/2
  [manche_actif] -> "Choix : accélération"/2
  "Manche : filtre du second ordre"/4(actif) -> [manche_actif]  "manche_actif"
  "Manche : filtre du second ordre"/1(angle) -> "Choix : angle"/1
  "Manche : filtre du second ordre"/2(vitesse) -> "Choix : vitesse"/1
  "Programme : polynômes de degré 5"/2(vitesse) -> "Choix : vitesse"/3
  "Manche : filtre du second ordre"/3(acceleration) -> "Choix : accélération"/1
  "Programme : polynômes de degré 5"/3(acceleration) -> "Choix : accélération"/3
  "Choix : angle"/1 -> Consigne/1  "angles_ref_deg"
  "Choix : vitesse"/1 -> Consigne/2  "vitesses_ref_dps"
  "Choix : accélération"/1 -> Consigne/3  "accelerations_ref_dps2"
  Consigne/1 -> consigne (°)/1

== system jumeau_banc_rw/Tableau de bord ==
  note: Tableau de bord : l'état du banc envoyé à l'interface de pilotage toutes les T_affichage secondes (0,1 s).
      | Il n'utilise que l'état donné par la Perception : il marchera de la même façon avec le banc réel.
  état : Inport
  consigne : Inport  Port=2
  poussée (N.m) : Inport  Port=3
  Consigne : BusSelector  OutputSignals=angles_ref_deg
  Envoi à l'interface : MATLAB Function  TreatAsAtomicUnit=on
  Temps : DigitalClock  SampleTime=T_affichage
  État : BusSelector  OutputSignals=angles_deg,vitesses_roues,reserve_roues,desequilibre_mm
  wires:
  état/1 -> État/1
  consigne/1 -> Consigne/1
  État/1 -> Envoi à l'interface/1(angles_deg)  "<angles_deg>"
  État/2 -> Envoi à l'interface/2(roues)  "<vitesses_roues>"
  État/3 -> Envoi à l'interface/3(reserve)  "<reserve_roues>"
  État/4 -> Envoi à l'interface/4(desequilibre_mm)  "<desequilibre_mm>"
  Consigne/1 -> Envoi à l'interface/5(reference_deg)  "<angles_ref_deg>"
  poussée (N.m)/1 -> Envoi à l'interface/6(poussee)
  Temps/1 -> Envoi à l'interface/7(t)

== system jumeau_banc_rw/Commande bas niveau/+ consigne d'essai ==
  note: Consigne d'essai, ajoutée à la consigne qui vient de la conversion : deux paliers de vitesse reliés par des rampes.
      | Réglages dans le Model Workspace : essai_roue_t1, essai_roue_vitesse1, essai_roue_t2, essai_roue_vitesse2, essai_roue_acc.
      | La pente de la rampe donne l'accélération de référence. Pour ne rien ajouter : mettre les deux paliers à [0 0 0 0].
  vitesse demandée (rad par s) : Inport
  accélération demandée (rad par s²) : Inport  Port=2
  + accélération d'essai : Sum
  + vitesse d'essai : Sum
  Lecture de l'accélération : ZeroOrderHold  SampleTime=T_cbn
  Lecture de la vitesse : ZeroOrderHold  SampleTime=T_cbn
  Palier 1 : Step  Time=essai_roue_t1  Before=[0; 0; 0; 0]  After=essai_roue_vitesse1(:)  SampleTime=T_cbn
  Palier 2 : Step  Time=essai_roue_t2  Before=[0; 0; 0; 0]  After=essai_roue_vitesse2(:) - essai_roue_vitesse1(:)  SampleTime=T_cbn
  Paliers : Sum
  Pente de la rampe : simulink/Discrete/Discrete Derivative  gainval=1.0  ICPrevScaledInput=0.0  OutMin=[]  OutMax=[]  OutDataType=fixdt(1, 16)  OutScaling=2^-10  DoSatur=off
  Rampe : RateLimiter  RisingSlewLimit=essai_roue_acc  FallingSlewLimit=-essai_roue_acc  SampleTimeMode=inherited
  omega de référence (rad par s) : Outport
  accélération de référence (rad par s²) : Outport  Port=2
  wires:
  vitesse demandée (rad par s)/1 -> Lecture de la vitesse/1
  accélération demandée (rad par s²)/1 -> Lecture de l'accélération/1
  Lecture de la vitesse/1 -> + vitesse d'essai/1
  Lecture de l'accélération/1 -> + accélération d'essai/1
  [vitesse_essai] -> + vitesse d'essai/2
  [acceleration_essai] -> + accélération d'essai/2
  + vitesse d'essai/1 -> omega de référence (rad par s)/1
  + accélération d'essai/1 -> accélération de référence (rad par s²)/1
  Palier 1/1 -> Paliers/1
  Palier 2/1 -> Paliers/2
  Paliers/1 -> Rampe/1
  Rampe/1 -> [vitesse_essai], Pente de la rampe/1  "vitesse_essai"
  Pente de la rampe/1 -> [acceleration_essai]  "acceleration_essai"

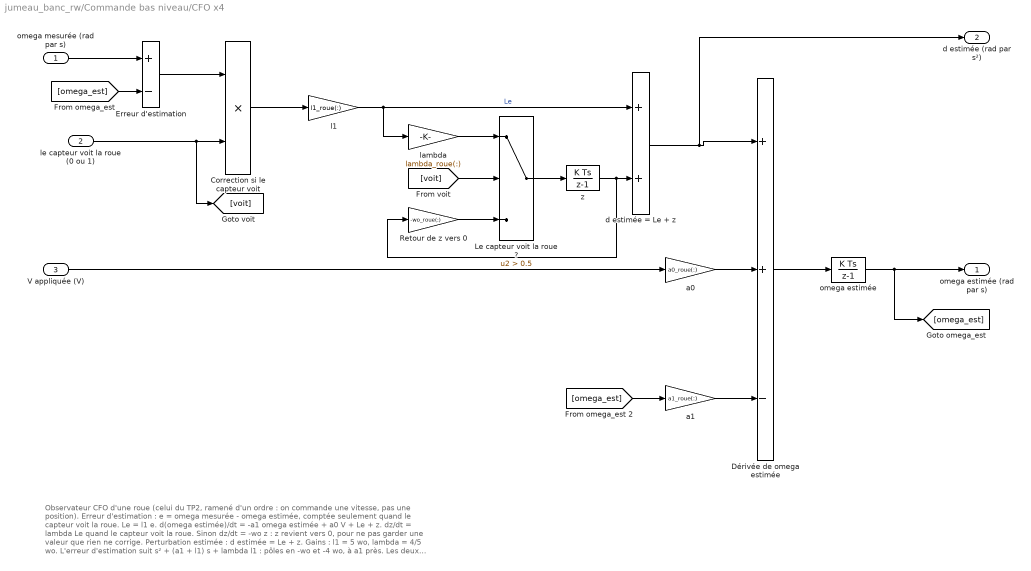
== system jumeau_banc_rw/Commande bas niveau/CFO x4 ==
  note: Observateur CFO d'une roue (celui du TP2, ramené d'un ordre : on commande une vitesse, pas une position).
      | Erreur d'estimation : e = omega mesurée - omega estimée, comptée seulement quand le capteur voit la roue.          Le = l1 e.
      | d(omega estimée)/dt = -a1 omega estimée + a0 V + Le + z.
      | dz/dt = lambda Le quand le capteur voit la roue. Sinon dz/dt = -wo z : z revient vers 0, pour ne pas garder une valeur que rien ne corrige.
      | Perturbation estimée : d estimée = Le + z.
      | Gains : l1 = 5 wo, lambda = 4/5 wo. L'erreur d'estimation suit s² + (a1 + l1) s + lambda l1 : pôles en -wo et -4 wo, à a1 près.
      | Les deux intégrateurs sont discrets (Euler, période T_cbn).
  omega mesurée (rad par s) : Inport
  le capteur voit la roue (0 ou 1) : Inport  Port=2
  V appliquée (V) : Inport  Port=3
  Correction si le capteur voit : Product
  Dérivée de omega estimée : Sum  Inputs=++-
  Erreur d'estimation : Sum  Inputs=+-
  Le capteur voit la roue ? : Switch  Criteria=u2 > Threshold  Threshold=0.5  SaturateOnIntegerOverflow=off  InputSameDT=off
  Retour de z vers 0 : Gain  Gain=-wo_roue(:)
  a0 : Gain  Gain=a0_roue(:)
  a1 : Gain  Gain=a1_roue(:)
  d estimée = Le + z : Sum
  l1 : Gain  Gain=l1_roue(:)
  lambda : Gain  Gain=lambda_roue(:)
  omega estimée : DiscreteIntegrator  gainval=1  SampleTime=T_cbn  ICPrevOutput=DiscIntNeverNeededParam  ICPrevScaledInput=DiscIntNeverNeededParam
  z : DiscreteIntegrator  gainval=1  SampleTime=T_cbn  ICPrevOutput=DiscIntNeverNeededParam  ICPrevScaledInput=DiscIntNeverNeededParam
  omega estimée (rad par s) : Outport
  d estimée (rad par s²) : Outport  Port=2
  wires:
  omega mesurée (rad par s)/1 -> Erreur d'estimation/1
  [omega_est] -> Erreur d'estimation/2
  Erreur d'estimation/1 -> Correction si le capteur voit/1
  le capteur voit la roue (0 ou 1)/1 -> Correction si le capteur voit/2, [voit]
  Correction si le capteur voit/1 -> l1/1
  l1/1 -> d estimée = Le + z/1, lambda/1  "Le"
  lambda/1 -> Le capteur voit la roue ?/1
  [voit] -> Le capteur voit la roue ?/2
  Retour de z vers 0/1 -> Le capteur voit la roue ?/3
  Le capteur voit la roue ?/1 -> z/1
  z/1 -> d estimée = Le + z/2, Retour de z vers 0/1
  d estimée = Le + z/1 -> Dérivée de omega estimée/1, d estimée (rad par s²)/1
  V appliquée (V)/1 -> a0/1
  a0/1 -> Dérivée de omega estimée/2
  [omega_est] -> a1/1
  a1/1 -> Dérivée de omega estimée/3
  Dérivée de omega estimée/1 -> omega estimée/1
  omega estimée/1 -> omega estimée (rad par s)/1, [omega_est]

== system jumeau_banc_rw/Commande bas niveau/Interface tension - impulsion x4 ==
  note: Interface tension - impulsion : l'ESC applique V = V_alim (impulsion - neutre) / (imp_max - imp_neutre), dans le sens de rotation du moteur.
      | L'impulsion est bornée de imp_cmd_min à imp_cmd_max (vitesse conseillée des disques) et arrondie à 1 µs, comme dans la trame de commande.
      | Seconde sortie : la tension réellement appliquée, recalculée à partir de l'impulsion envoyée. C'est elle que le CFO doit recevoir.
  V commandée (V) : Inport
  + neutre : Bias  Bias=imp_neutre  SaturateOnIntegerOverflow=off
  - neutre : Bias  Bias=-imp_neutre  SaturateOnIntegerOverflow=off
  Arrondi à 1 µs : Rounding  Operator=round
  Limites des disques : Saturate  UpperLimit=imp_cmd_max  LowerLimit=imp_cmd_min
  Sens de rotation : Gain  Gain=sens_moteurs(:)
  Sens de rotation (retour) : Gain  Gain=sens_moteurs(:)
  Volts vers µs : Gain  Gain=(imp_max - imp_neutre)/V_alim
  µs vers volts : Gain  Gain=V_alim/(imp_max - imp_neutre)
  impulsions (µs) : Outport
  V appliquée (V) : Outport  Port=2
  wires:
  V commandée (V)/1 -> Volts vers µs/1
  Volts vers µs/1 -> Sens de rotation/1
  Sens de rotation/1 -> + neutre/1
  + neutre/1 -> Limites des disques/1
  Limites des disques/1 -> Arrondi à 1 µs/1
  Arrondi à 1 µs/1 -> impulsions (µs)/1, [impulsions]
  [impulsions] -> - neutre/1
  - neutre/1 -> Sens de rotation (retour)/1
  Sens de rotation (retour)/1 -> µs vers volts/1
  µs vers volts/1 -> V appliquée (V)/1

== system jumeau_banc_rw/Commande bas niveau/Loi de commande x4 ==
  note: Loi de commande d'une roue (celle du TP2, ramenée à la vitesse).
      | Erreur de suivi : e = omega estimée - omega de référence. Commande virtuelle : -K e, avec K = wc - a1. L'erreur suit alors de/dt = -wc e.
      | Tension : V = (-K e - d estimée + a1 omega de référence + accélération de référence) / a0.
  omega de référence (rad par s) : Inport
  accélération de référence (rad par s²) : Inport  Port=2
  omega estimée (rad par s) : Inport  Port=3
  d estimée (rad par s²) : Inport  Port=4
  1 sur a0 : Gain  Gain=1./a0_roue(:)
  Erreur de suivi : Sum  Inputs=+-
  K : Gain  Gain=K_roue(:)
  Somme : Sum  Inputs=++--
  a1 : Gain  Gain=a1_roue(:)
  V commandée (V) : Outport
  wires:
  omega de référence (rad par s)/1 -> a1/1, [omega_ref]
  a1/1 -> Somme/1
  accélération de référence (rad par s²)/1 -> Somme/2
  omega estimée (rad par s)/1 -> Erreur de suivi/1
  [omega_ref] -> Erreur de suivi/2
  Erreur de suivi/1 -> K/1
  K/1 -> Somme/3
  d estimée (rad par s²)/1 -> Somme/4
  Somme/1 -> 1 sur a0/1
  1 sur a0/1 -> V commandée (V)/1

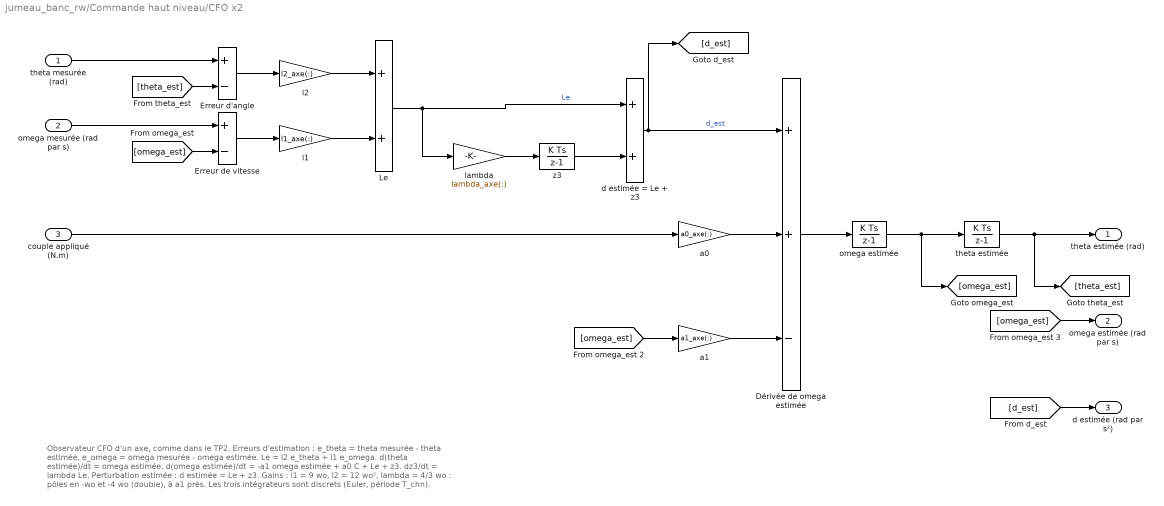
== system jumeau_banc_rw/Commande haut niveau/CFO x2 ==
  note: Observateur CFO d'un axe, comme dans le TP2.
      | Erreurs d'estimation : e_theta = theta mesurée - theta estimée, e_omega = omega mesurée - omega estimée.          Le = l2 e_theta + l1 e_omega.
      | d(theta estimée)/dt = omega estimée.
      | d(omega estimée)/dt = -a1 omega estimée + a0 C + Le + z3.
      | dz3/dt = lambda Le.
      | Perturbation estimée : d estimée = Le + z3.
      | Gains : l1 = 9 wo, l2 = 12 wo², lambda = 4/3 wo : pôles en -wo et -4 wo (double), à a1 près.
      | Les trois intégrateurs sont discrets (Euler, période T_chn).
  theta mesurée (rad) : Inport
  omega mesurée (rad par s) : Inport  Port=2
  couple appliqué (N.m) : Inport  Port=3
  Dérivée de omega estimée : Sum  Inputs=++-
  Erreur d'angle : Sum  Inputs=+-
  Erreur de vitesse : Sum  Inputs=+-
  Le : Sum
  a0 : Gain  Gain=a0_axe(:)
  a1 : Gain  Gain=a1_axe(:)
  d estimée = Le + z3 : Sum
  l1 : Gain  Gain=l1_axe(:)
  l2 : Gain  Gain=l2_axe(:)
  lambda : Gain  Gain=lambda_axe(:)
  omega estimée : DiscreteIntegrator  gainval=1  SampleTime=T_chn  ICPrevOutput=DiscIntNeverNeededParam  ICPrevScaledInput=DiscIntNeverNeededParam
  theta estimée : DiscreteIntegrator  gainval=1  InitialCondition=q0_deg(:)*pi/180  SampleTime=T_chn  ICPrevOutput=DiscIntNeverNeededParam  ICPrevScaledInput=DiscIntNeverNeededParam
  z3 : DiscreteIntegrator  gainval=1  SampleTime=T_chn  ICPrevOutput=DiscIntNeverNeededParam  ICPrevScaledInput=DiscIntNeverNeededParam
  theta estimée (rad) : Outport
  omega estimée (rad par s) : Outport  Port=2
  d estimée (rad par s²) : Outport  Port=3
  wires:
  theta mesurée (rad)/1 -> Erreur d'angle/1
  [theta_est] -> Erreur d'angle/2
  omega mesurée (rad par s)/1 -> Erreur de vitesse/1
  [omega_est] -> Erreur de vitesse/2
  Erreur d'angle/1 -> l2/1
  Erreur de vitesse/1 -> l1/1
  l2/1 -> Le/1
  l1/1 -> Le/2
  Le/1 -> d estimée = Le + z3/1, lambda/1  "Le"
  lambda/1 -> z3/1
  z3/1 -> d estimée = Le + z3/2
  d estimée = Le + z3/1 -> Dérivée de omega estimée/1, [d_est]  "d_est"
  couple appliqué (N.m)/1 -> a0/1
  a0/1 -> Dérivée de omega estimée/2
  [omega_est] -> a1/1
  a1/1 -> Dérivée de omega estimée/3
  Dérivée de omega estimée/1 -> omega estimée/1
  omega estimée/1 -> theta estimée/1, [omega_est]
  theta estimée/1 -> theta estimée (rad)/1, [theta_est]
  [omega_est] -> omega estimée (rad par s)/1
  [d_est] -> d estimée (rad par s²)/1

== system jumeau_banc_rw/Commande haut niveau/Limite et mise en marche x2 ==
  note: Le couple est borné à C_max : au-delà, les roues devraient accélérer plus vite que acc_roue_max.
      | Avant t_depart, le couple demandé est nul : le dispositif est tenu à la main et les roues se mettent en rotation.
  couple calculé (N.m) : Inport
  Couple maximal : Saturate  UpperLimit=C_max  LowerLimit=-C_max
  Marche à t_depart : Step  Time=t_depart  SampleTime=T_chn
  x marche : Product
  couple appliqué (N.m) : Outport
  wires:
  couple calculé (N.m)/1 -> Couple maximal/1
  Couple maximal/1 -> x marche/1
  Marche à t_depart/1 -> x marche/2
  x marche/1 -> couple appliqué (N.m)/1

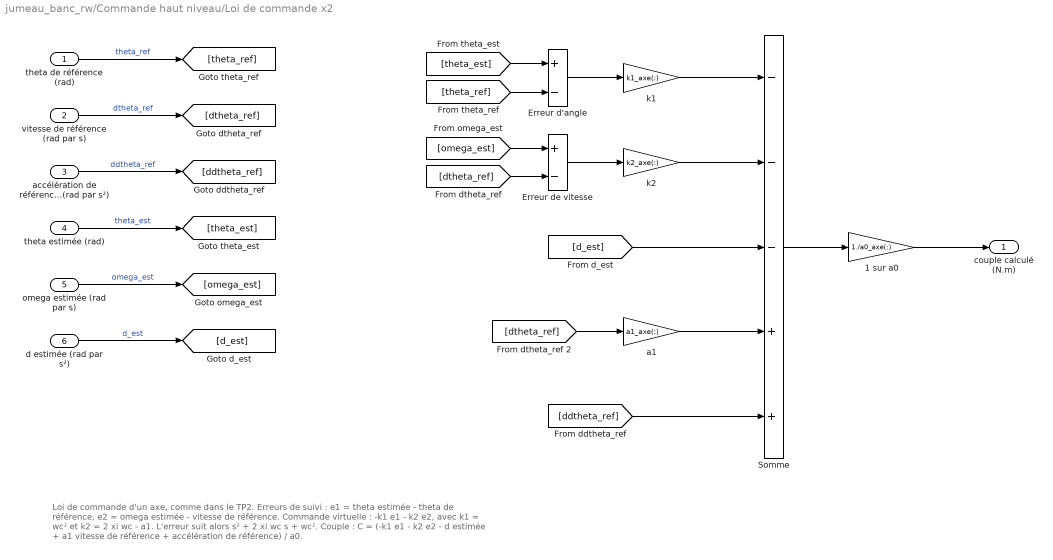
== system jumeau_banc_rw/Commande haut niveau/Loi de commande x2 ==
  note: Loi de commande d'un axe, comme dans le TP2.
      | Erreurs de suivi : e1 = theta estimée - theta de référence, e2 = omega estimée - vitesse de référence.
      | Commande virtuelle : -k1 e1 - k2 e2, avec k1 = wc² et k2 = 2 xi wc - a1. L'erreur suit alors s² + 2 xi wc s + wc².
      | Couple : C = (-k1 e1 - k2 e2 - d estimée + a1 vitesse de référence + accélération de référence) / a0.
  theta de référence (rad) : Inport
  vitesse de référence (rad par s) : Inport  Port=2
  accélération de référence (rad par s²) : Inport  Port=3
  theta estimée (rad) : Inport  Port=4
  omega estimée (rad par s) : Inport  Port=5
  d estimée (rad par s²) : Inport  Port=6
  1 sur a0 : Gain  Gain=1./a0_axe(:)
  Erreur d'angle : Sum  Inputs=+-
  Erreur de vitesse : Sum  Inputs=+-
  Somme : Sum  Inputs=---++
  a1 : Gain  Gain=a1_axe(:)
  k1 : Gain  Gain=k1_axe(:)
  k2 : Gain  Gain=k2_axe(:)
  couple calculé (N.m) : Outport
  wires:
  theta de référence (rad)/1 -> [theta_ref]  "theta_ref"
  vitesse de référence (rad par s)/1 -> [dtheta_ref]  "dtheta_ref"
  accélération de référence (rad par s²)/1 -> [ddtheta_ref]  "ddtheta_ref"
  theta estimée (rad)/1 -> [theta_est]  "theta_est"
  omega estimée (rad par s)/1 -> [omega_est]  "omega_est"
  d estimée (rad par s²)/1 -> [d_est]  "d_est"
  [theta_est] -> Erreur d'angle/1
  [theta_ref] -> Erreur d'angle/2
  [omega_est] -> Erreur de vitesse/1
  [dtheta_ref] -> Erreur de vitesse/2
  Erreur d'angle/1 -> k1/1
  Erreur de vitesse/1 -> k2/1
  k1/1 -> Somme/1
  k2/1 -> Somme/2
  [d_est] -> Somme/3
  [dtheta_ref] -> a1/1
  a1/1 -> Somme/4
  [ddtheta_ref] -> Somme/5
  Somme/1 -> 1 sur a0/1
  1 sur a0/1 -> couple calculé (N.m)/1

== system jumeau_banc_rw/Commande haut niveau/Mesures x2 ==
  note: Angles et vitesses de roulis et de tangage, donnés par la Perception (quaternion et gyroscope du BNO055, ramenés aux axes
      | du cardan), lus à chaque période de la commande.
  angles (rad) : Inport
  vitesses (rad par s) : Inport  Port=2
  Lecture des angles : ZeroOrderHold  SampleTime=T_chn
  Lecture des vitesses : ZeroOrderHold  SampleTime=T_chn
  theta mesurée (rad) : Outport
  omega mesurée (rad par s) : Outport  Port=2
  wires:
  angles (rad)/1 -> Lecture des angles/1
  Lecture des angles/1 -> theta mesurée (rad)/1
  vitesses (rad par s)/1 -> Lecture des vitesses/1
  Lecture des vitesses/1 -> omega mesurée (rad par s)/1

== system jumeau_banc_rw/Commande haut niveau/Référence et désaturation x2 ==
  note: La référence arrive en degrés et repart en radians.
      | Désaturation. Un couple constant sur un axe oblige les roues à accélérer sans fin. Le moment cinétique des roues est mesuré par la
      | Perception (vitesses des roues avec leur signe). La référence d'angle est décalée de k_desat fois ce moment : le dispositif se penche un peu, et la
      | pesanteur rend aux roues leur vitesse de repos avec la constante de temps T_desat. À la fin, le dispositif est à son point d'équilibre.
      | desat_active = 0 : pas de décalage. C'est le réglage du banc équilibré : il n'a plus de point d'équilibre imposé, et se pencher ne
      | décharge plus les roues.
  angle demandé (°) : Inport
  vitesse demandée (° par s) : Inport  Port=2
  accélération demandée (° par s²) : Inport  Port=3
  moment cinétique des roues (N.m.s) : Inport  Port=4
  Décalage maximal : Saturate  UpperLimit=desat_max_deg*pi/180  LowerLimit=-desat_max_deg*pi/180
  Lecture du moment : ZeroOrderHold  SampleTime=T_chn
  Référence décalée : Sum  Inputs=+-
  en radians 1 : Gain  Gain=pi/180
  en radians 2 : Gain  Gain=pi/180
  en radians 3 : Gain  Gain=pi/180
  k_desat : Gain  Gain=k_desat(:)
  theta de référence (rad) : Outport
  vitesse de référence (rad par s) : Outport  Port=2
  accélération de référence (rad par s²) : Outport  Port=3
  wires:
  angle demandé (°)/1 -> en radians 1/1
  vitesse demandée (° par s)/1 -> en radians 2/1
  accélération demandée (° par s²)/1 -> en radians 3/1
  en radians 1/1 -> Référence décalée/1
  [decalage] -> Référence décalée/2
  Référence décalée/1 -> theta de référence (rad)/1
  en radians 2/1 -> vitesse de référence (rad par s)/1
  en radians 3/1 -> accélération de référence (rad par s²)/1
  moment cinétique des roues (N.m.s)/1 -> Lecture du moment/1
  Lecture du moment/1 -> k_desat/1
  k_desat/1 -> Décalage maximal/1
  Décalage maximal/1 -> [decalage]  "decalage"

== system jumeau_banc_rw/Perception/Couple extérieur et déséquilibre x2 ==
  note: Couple extérieur sur le dispositif (pesanteur, poussées), sur [roulis ; tangage] : quand le dispositif est immobile, c'est le couple que
      | les roues absorbent, la dérivée de leur moment cinétique. Il est filtré par un premier ordre de constante de temps tau_desequilibre.
      | Déséquilibre : le couple de pesanteur vaut m g fois le décalage horizontal du centre de masse. On en tire la position du centre de
      | masse par rapport au pivot, en mm, [selon X ; selon Y] : x = couple de tangage / (m g), y = -couple de roulis / (m g).
      | C'est le réglage à reporter sur les écrous d'équilibrage. Juste pendant que le dispositif est immobile.
  moment cinétique (N.m.s) : Inport
  1 sur tau : Gain  Gain=1/tau_desequilibre
  H - H filtré : Sum  Inputs=+-
  H filtré : DiscreteIntegrator  gainval=1  SampleTime=T_perception  ICPrevOutput=DiscIntNeverNeededParam  ICPrevScaledInput=DiscIntNeverNeededParam
  vers le centre de masse : Gain  Gain=1000/max(g, 0.01)*[0 1/m_disp; -1/(m_disp + m_croix) 0]  Multiplication=Matrix(K*u)
  couple extérieur (N.m) : Outport
  déséquilibre (mm) : Outport  Port=2
  wires:
  moment cinétique (N.m.s)/1 -> H - H filtré/1
  H - H filtré/1 -> 1 sur tau/1
  1 sur tau/1 -> H filtré/1, couple extérieur (N.m)/1, vers le centre de masse/1
  H filtré/1 -> H - H filtré/2
  vers le centre de masse/1 -> déséquilibre (mm)/1

== system jumeau_banc_rw/Perception/Inclinaison x2 ==
  note: Angles du cardan, tirés du quaternion du BNO055 : pas de 2^-14, contre 1/16° pour les angles d'Euler, et exacts quand le
      | roulis et le tangage se combinent (les angles d'Euler du capteur suivent la séquence Z-Y-X, pas celle du cardan).
      | Vitesses de roulis et de tangage, tirées du gyroscope et des angles. Le cap du capteur n'intervient pas.
  quaternion : Inport
  gyroscope (° par s) : Inport  Port=2
  Angles du cardan (quaternion) : MATLAB Function  TreatAsAtomicUnit=on
  Lecture du gyroscope : ZeroOrderHold  SampleTime=T_perception
  Lecture du quaternion : ZeroOrderHold  SampleTime=T_perception
  Vitesses du cardan (gyroscope) : MATLAB Function  TreatAsAtomicUnit=on
  angles (rad) : Outport
  vitesses (rad par s) : Outport  Port=2
  wires:
  quaternion/1 -> Lecture du quaternion/1
  Lecture du quaternion/1 -> Angles du cardan (quaternion)/1(q)
  gyroscope (° par s)/1 -> Lecture du gyroscope/1
  Lecture du gyroscope/1 -> Vitesses du cardan (gyroscope)/1(gyro_dps)
  Angles du cardan (quaternion)/1(angles) -> angles (rad)/1, Vitesses du cardan (gyroscope)/2(angles)
  Vitesses du cardan (gyroscope)/1(vitesses) -> vitesses (rad par s)/1

== system jumeau_banc_rw/Perception/Moment cinétique des roues x2 ==
  note: Moment cinétique des 4 roues par rapport au dispositif, sur [roulis ; tangage] : H = J cos 45° [somme sx w ; somme sy w].
      | À la vitesse de repos, les 4 roues s'annulent deux à deux : H = 0.
  vitesses des roues (rad par s) : Inport
  J cos 45° [sx ; sy] : Gain  Gain=J_roue*cosd(45)*[sx_roues; sy_roues]  Multiplication=Matrix(K*u)
  moment cinétique (N.m.s) : Outport
  wires:
  vitesses des roues (rad par s)/1 -> J cos 45° [sx ; sy]/1
  J cos 45° [sx ; sy]/1 -> moment cinétique (N.m.s)/1

== system jumeau_banc_rw/Perception/Réserve des roues ==
  vitesses des roues (rad par s) : Inport
  Marge aux limites : MATLAB Function  TreatAsAtomicUnit=on
  réserve (0 à 1) : Outport
  wires:
  vitesses des roues (rad par s)/1 -> Marge aux limites/1(w)
  Marge aux limites/1(r) -> réserve (0 à 1)/1
